simulink model "BEV_Thermal_Management"  (R2025a)
settings: Solver=ode23t  StartTime=0  StopTime=765  MaxStep=5  RelTol=1e-3  AbsTol=1e-3
model workspace: external: MATLAB File BEV_Thermal_Management_param.m (data not in the file)
undefined symbols (not defined in the file): Battery, bulb, cabin_doors_conductivity, cabin_duct_area, cabin_glass_conductivity, cabin_roof_conductivity, cabin_T_init, chiller_area_primary, chiller_N_baffles, chiller_N_tubes, chiller_tube_D, chiller_tube_L, chiller_wall_conductivity, chiller_wall_thickness, compressor_rpm_LUT, condenser_air_area_flow, condenser_air_area_primary, condenser_W, condenser_wall_conductivity, condenser_wall_thickness, coolant_channel_D, coolant_pipe_area, coolant_pipe_D, coolant_T_init, coolant_tank_area, coolant_tank_volume, coolant_valve_D_ratio_max, coolant_valve_D_ratio_min, coolant_valve_displacement, coolant_valve_S_max, cycle, DCDC, Edrive, evaporator_air_area_flow, evaporator_air_area_primary, evaporator_W, evaporator_wall_conductivity, evaporator_wall_thickness, heater_max_power, ModuleType1, outlet, ptc_max_power, pump_speed_max, radiationReflectionShields, radiator_air_area_flow, radiator_air_area_primary, radiator_W, radiator_wall_conductivity, radiator_wall_thickness, refrigerant_alpha_init, refrigerant_pipe_D, transRatio
libraries: fl_lib x264, nesl_utility x91, SimscapeFluids_lib x22, sdl_lib x13, ee_lib x9, nesl_utility_internal x4, slpidlib x3, BatteryProtection x3, batt_lib x2, BatteryCurrentManagement x1, autolibsharedcommon x1, simulink x1
(part 3 of 9)

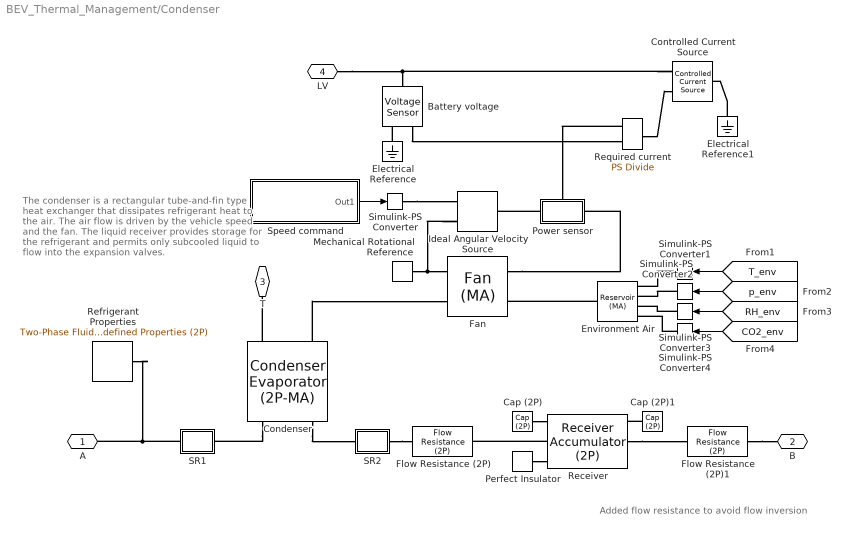
== system BEV_Thermal_Management/Condenser ==
  note: Added flow resistance to avoid flow inversion
  note: The condenser is a rectangular tube-and-fin type heat exchanger that dissipates refrigerant heat to the air. The air flow is driven by the vehicle speed and the fan. The liquid receiver provides storage for the refrigerant and permits only subcooled liquid to flow into the expansion valves.
  Battery voltage : fl_lib/Electrical/Electrical Sensors/Voltage Sensor
  Cap (2P) : fl_lib/Two-Phase Fluid/Elements/Cap (2P)  p_specify=off  p_priority=None  p=0.101325 MPa  p_nominal_specify=off  p_nominal_value=1  p_nominal_unit=MPa  u_specify=off  u_priority=None  u=1.5e+3 kJ/kg  u_nominal_specify=off  u_nominal_value=1  u_nominal_unit=kJ/kg
      settings: InternalSimscapePortConfiguration="{\"Bottom\":[],\"Left\":[{\"id\":\"A\",\"label\":\"\",\"type\":\"foundation.two_phase_fluid.two_phase_fluid\"}],\"Right\":[],\"Top\":[]}"
  Cap (2P)1 : fl_lib/Two-Phase Fluid/Elements/Cap (2P)  p_specify=off  p_priority=None  p=0.101325 MPa  p_nominal_specify=off  p_nominal_value=1  p_nominal_unit=MPa  u_specify=off  u_priority=None  u=1.5e+3 kJ/kg  u_nominal_specify=off  u_nominal_value=1  u_nominal_unit=kJ/kg
      settings: InternalSimscapePortConfiguration="{\"Bottom\":[],\"Left\":[{\"id\":\"A\",\"label\":\"\",\"type\":\"foundation.two_phase_fluid.two_phase_fluid\"}],\"Right\":[],\"Top\":[]}"
  Condenser : SimscapeFluids_lib/Heat Exchangers/Two-Phase Fluid - Moist Air/Condenser Evaporator (2P-MA)  flow_arrangement=fluids.heat_exchangers.enum.FlowArrangement2PMA.Cross  cross_flow_arrangement=fluids.heat_exchangers.enum.CrossFlowArrangement2PMA.UnmixedUnmixed  R_wall=condenser_wall_thickness / condenser_air_area_primary / condenser_wall_conductivity K/W  wall_thermal_mass=false  mass_wall=1 kg  cp_wall=490 J/(K*kg)  area_A1=pi * refrigerant_pipe_D^2 / 4 m^2  area_B1=pi * refrigerant_pipe_D^2 / 4 m^2  area_A2=cabin_duct_area m^2  area_B2=cabin_duct_area m^2  tube_num_2P=condenser_N_tubes  tube_length_2P=condenser_L m  tube_cross_section_2P=fluids.heat_exchangers.enum.TubeCrossSection.Rectangular  tube_diameter_2P=0.1 m  tube_width_2P=condenser_W m  tube_height_2P=condenser_tube_H m  tube_inner_diameter_2P=0.05 m  tube_outer_diameter_2P=0.1 m  tube_flow_area_2P=0.01 m^2  tube_wetted_perimeter_2P=0.4 m  tube_heat_perimeter_2P=0.4 m  tube_pressure_loss_spec_2P=fluids.heat_exchangers.enum.TubePressureLossSpec2P.Haaland  tube_loss_coeff_2P=10  tube_local_pressure_loss_spec_2P=fluids.heat_exchangers.enum.LocalLossSpec.AggregateLength  tube_length_add_2P=condenser_tube_Leq m  tube_local_loss_coefficient_2P=0.1  tube_roughness_pressure_2P=15e-6 m  tube_Re_lam_pressure_2P=2000  tube_Re_tur_pressure_2P=4000  tube_shape_factor_generic_2P=64  tube_heat_coeff_spec_2P=fluids.heat_exchangers.enum.TubeHeatCoeffSpec2P.GneilinskiCavalliniZecchin  tube_colburn_coeff_liq_2P=[.023, .8, .33]  tube_colburn_coeff_mix_2P=[.05, .8, .33]  tube_colburn_coeff_vap_2P=[.023, .8, .33]  tube_roughness_heat_2P=15e-6 m  tube_Re_lam_heat_2P=2000  tube_Re_tur_heat_2P=4000  tube_Nu_lam_generic_2P=3.66  fouling_factor_2P=0.1 m^2*K/kW  fin_area_2P=condenser_tube_area_webs m^2  fin_efficiency_2P=0.6  energy_spec_2P=foundation.enum.energy_spec.void_fraction  p_init_2P=refrigerant_p_init MPa  T_init_2P=293.15 K  x_init_2P=0.5  alpha_init_2P=refrigerant_alpha_init  h_init_2P=1500 kJ/kg  u_init_2P=1500 kJ/kg  flow_geometry_MA=fluids.heat_exchangers.enum.FlowGeometryMA.Generic  tube_num_MA=1  tube_length_MA=5 m  tube_cross_section_MA=fluids.heat_exchangers.enum.TubeCrossSection.Circular  tube_diameter_MA=0.1 m  tube_width_MA=0.1 m  tube_height_MA=0.1 m  tube_inner_diameter_MA=0.05 m  tube_outer_diameter_MA=0.1 m  tube_flow_area_MA=0.01 m^2  tube_wetted_perimeter_MA=0.4 m  tube_heat_perimeter_MA=0.4 m  tube_pressure_loss_spec_MA=fluids.heat_exchangers.enum.TubePressureLossSpec.Haaland  tube_loss_coeff_MA=10  tube_local_pressure_loss_spec_MA=fluids.heat_exchangers.enum.LocalLossSpec.AggregateLength  tube_length_add_MA=0.1 m  tube_local_loss_coefficient_MA=0.1  tube_roughness_pressure_MA=15e-6 m  tube_Re_lam_pressure_MA=2000  tube_Re_tur_pressure_MA=4000  tube_shape_factor_generic_MA=64  tube_heat_coeff_spec_MA=fluids.heat_exchangers.enum.TubeHeatCoeffSpec.Gneilinski  tube_colburn_coeff_MA=[.023, .8, .33]  tube_roughness_heat_MA=15e-6 m  tube_Re_lam_heat_MA=2000  tube_Re_tur_heat_MA=4000  tube_Nu_lam_generic_MA=3.66  bank_arrangement_MA=fluids.heat_exchangers.enum.BankArrangement.Inline  bank_num_rows_MA=5  bank_tubes_per_row_MA=5  bank_width_MA=1 m  bank_tube_diameter_MA=0.05 m  bank_longitudinal_pitch_MA=0.15 m  bank_transverse_pitch_MA=0.15 m  bank_pressure_loss_spec_MA=fluids.heat_exchangers.enum.BankPressureLossSpec.Martin  bank_euler_MA=10  bank_heat_coeff_spec_MA=fluids.heat_exchangers.enum.BankHeatCoeffSpec.Martin  bank_colburn_coeff_MA=[.27, .63, .36]  generic_flow_area_MA=condenser_air_area_flow m^2  generic_heat_area_MA=condenser_air_area_primary m^2  generic_volume_MA=condenser_air_area_flow * condenser_W m^3  generic_loss_coeff_MA=10  generic_colburn_coeff_MA=[0.27, 0.63, 0.36]  fouling_factor_MA=0.1 m^2*K/kW  fin_area_MA=condenser_air_area_fins m^2  fin_efficiency_MA=0.7  p_init_MA=cabin_p_init MPa  T_init_MA=cabin_T_init K  humidity_spec_MA=foundation.enum.HumiditySpec.RelativeHumidity  RH_init_MA=cabin_RH_init  x_w_init_MA=0.01  y_w_init_MA=0.01  HR_init_MA=0.01  Tw_init_MA=287 K  trace_gas_spec_MA=foundation.enum.trace_gas_spec.mole_fraction  x_g_init_MA=0.001  y_g_init_MA=cabin_CO2_init  r_d_init_MA=0  RH_ws_MA=1  time_constant_cond_MA=1e-3 s  time_constant_evap_MA=1e-3 s  fraction_entrained_MA=1
      settings: InternalSimscapePortConfiguration="{\"Bottom\":[],\"Left\":[{\"id\":\"A1\",\"label\":\"A1\",\"type\":\"foundation.two_phase_fluid.two_phase_fluid\"},{\"id\":\"Z\",\"label\":\"Z\",\"type\":\"output\"},{\"id\":\"B1\",\"label\":\"B1\",\"type\":\"foundation.two_phase_fluid.two_phase_fluid\"}],\"Right\":[{\"id\":\"A2\",\"label\":\"A2\",\"type\":\"foundation.moist_air.moist_air\"},{\"id\":\"W\",\"label\":\"W\",\"type\":\"output\"},{\"id\":\"B2\",\"label\":\"B2\",\"type\":\"foundation.moist_air.moist_air\"}],\"Top\":[]}"
  Controlled Current Source : fl_lib/Electrical/Electrical Sources/Controlled Current Source
  Electrical Reference : fl_lib/Electrical/Electrical Elements/Electrical Reference
  Electrical Reference1 : fl_lib/Electrical/Electrical Elements/Electrical Reference
  Environment Air : fl_lib/Moist Air/Elements/Reservoir (MA)  pressure_input=true  pressure_spec=foundation.enum.pressure_spec.atmospheric  reservoir_pressure=0.101325 MPa  temperature_input=true  temperature_spec=foundation.enum.temperature_spec.atmospheric  reservoir_temperature=293.15 K  humidity_input=true  humidity_spec=foundation.enum.HumiditySpec.RelativeHumidity  reservoir_RH=0.5  reservoir_x_w=0.01  reservoir_y_w=0.01  reservoir_HR=0.01  reservoir_Tw=287 K  trace_gas_input=true  trace_gas_spec=foundation.enum.trace_gas_spec.mole_fraction  reservoir_x_g=0.001  reservoir_y_g=0.001  water_droplets_input=false  reservoir_r_d=0  RH_ws=1  area_A=cabin_duct_area m^2  input_error_spec=foundation.enum.input_range_error.warn
      settings: InternalSimscapePortConfiguration="{\"Bottom\":[],\"Left\":[{\"id\":\"A\",\"label\":\"A\",\"type\":\"foundation.moist_air.moist_air\"}],\"Right\":[{\"id\":\"T\",\"label\":\"T\",\"type\":\"input\"},{\"id\":\"P\",\"label\":\"P\",\"type\":\"input\"},{\"id\":\"W\",\"label\":\"W\",\"type\":\"input\"},{\"id\":\"G\",\"label\":\"G\",\"type\":\"input\"}],\"Top\":[]}"
  Fan : SimscapeFluids_lib/Moist Air/Turbomachinery/Fan (MA)  fan_parameterization=fluids.moist_air.turbomachinery.enum.FanParameterization.Nominal  mechanical_power_spec=fluids.moist_air.turbomachinery.enum.FanMechanicalPowerSpec.Efficiency  flow_rate_nominal=0.8 m^3/s  pressure_nominal=400 Pa  eta_nominal=0.6  power_nominal=1620 W  pressure_max=600 Pa  flow_rate_max=1.5 m^3/s  omega_ref_nominal=1000 rpm  flow_rate_1D_TLU=[.0278, .0556, .0833, .111, .139, .167] m^3/s  pressure_1D_TLU=[6410, 6375, 6018, 5366, 4501, 3609] Pa  eta_1D_TLU=[.257, .394, .453, .47, .459, .415]  power_1D_TLU=[693, 900, 1107, 1267, 1363, 1452] W  omega_ref_1D=3000 rpm  rho_ref_1D=1.2 kg/m^3  omega_threshold_factor=1e-2  omega_dp_TLU=[2400; 3000; 3600] rpm  flow_rate_dp_TLU=[.0278, .0556, .0833, .111, .139, .167] m^3/s  pressure_dp_TLU=[4111, 4010, 3551, 2881, 2167, 1453; 6410, 6375, 6018, 5366, 4501, 3609; 9217, 9285, 9022, 8428, 7552, 6482] Pa  eta_dp_TLU=[.3, .434, .468, .459, .4, .3; .257, .394, .453, .47, .459, .415; .225, .359, .434, .461, .47, .459]  power_dp_TLU=[381, 514, 632, 697, 753, 809; 693, 900, 1107, 1267, 1363, 1452; 1139, 1438, 1732, 2029, 2233, 2358] W  rho_ref_dp=1.2 kg/m^3  omega_q_TLU=[2990; 3450; 3867] rpm  pressure_q_TLU=[31, 62, 93, 124] Pa  flow_rate_q_TLU=[.802, .759, .703, .611; .936, .902, .862, .81; 1.056, 1.027, .994, .956] m^3/s  eta_q_TLU=[.088, .162, .22, .261; .068, .128, .18, .222; .055, .105, .148, .188]  power_q_TLU=[283, 290, 297, 290; 427, 437, 445, 452; 595, 606, 625, 631] W  rho_ref_q=1.2 kg/m^3  diameter_ratio=1  mech_orientation=fluids.moist_air.turbomachinery.enum.FanMechanicalOrientation.Positive  area_A=cabin_duct_area m^2  area_B=cabin_duct_area m^2
      settings: InternalSimscapePortConfiguration="{\"Bottom\":[],\"Left\":[{\"id\":\"A\",\"label\":\"A\",\"type\":\"foundation.moist_air.moist_air\"},{\"id\":\"C\",\"label\":\"C\",\"type\":\"foundation.mechanical.rotational.rotational\"}],\"Right\":[{\"id\":\"B\",\"label\":\"B\",\"type\":\"foundation.moist_air.moist_air\"},{\"id\":\"R\",\"label\":\"R\",\"type\":\"foundation.mechanical.rotational.rotational\"}],\"Top\":[]}"
  Flow Resistance (2P) : fl_lib/Two-Phase Fluid/Elements/Flow Resistance (2P)  delta_p_nominal=1e-2 MPa  mdot_nominal=0.01 kg/s  v_nominal=0 m^3/kg  area=pi * refrigerant_pipe_D^2 / 4 m^2  laminar_fraction=1e-3
      settings: InternalSimscapePortConfiguration="{\"Bottom\":[],\"Left\":[{\"id\":\"A\",\"label\":\"A\",\"type\":\"foundation.two_phase_fluid.two_phase_fluid\"}],\"Right\":[{\"id\":\"B\",\"label\":\"B\",\"type\":\"foundation.two_phase_fluid.two_phase_fluid\"}],\"Top\":[]}"
  Flow Resistance (2P)1 : fl_lib/Two-Phase Fluid/Elements/Flow Resistance (2P)  delta_p_nominal=1e-2 MPa  mdot_nominal=0.01 kg/s  v_nominal=0 m^3/kg  area=pi * refrigerant_pipe_D^2 / 4 m^2  laminar_fraction=1e-3
      settings: InternalSimscapePortConfiguration="{\"Bottom\":[],\"Left\":[{\"id\":\"A\",\"label\":\"A\",\"type\":\"foundation.two_phase_fluid.two_phase_fluid\"}],\"Right\":[{\"id\":\"B\",\"label\":\"B\",\"type\":\"foundation.two_phase_fluid.two_phase_fluid\"}],\"Top\":[]}"
  Ideal Angular Velocity Source : fl_lib/Mechanical/Mechanical Sources/Ideal Angular Velocity Source
  Mechanical Rotational Reference : fl_lib/Mechanical/Rotational Elements/Mechanical Rotational Reference
  Perfect Insulator : fl_lib/Thermal/Thermal Elements/Perfect Insulator  T_specify=off  T_priority=None  T=0 K  T_nominal_specify=off  T_nominal_value=1  T_nominal_unit=K
  Power sensor : Subsystem
      settings: PortSchema="{\"entries\":[{\"content\":{\"sides\":[{\"content\":{\"connectorIds\":[\"LConn1\"]},\"type\":\"ConnectorPlacement.EquallySpacedRectSide\",\"uuid\":\"14aacb84-4d2c-4fe3-9667-966fc9affdc2\"},{\"content\":{\"connectorIds\":[\"RConn1\"],\"side\":\"RIGHT\"},\"type\":\"ConnectorPlacement.EquallySpacedRectSide\",\"uuid\":\"5f04cc75-bf75-44ff-ad13-d2b18990cf19\"},{\"content\":{\"connectorIds\":[\"LConn2\"],\"side\":\"TOP\"},\"type\":\"ConnectorPlacement.EquallySpacedRectSide\",\"uuid\":\"fdf9b4dd-6b03-4f92-a45a-c9cb867bd95a\"}]},\"type\":\"ConnectorPlacement.EquallySpacedConnector\",\"uuid\":\"3effddba-6f65-4497-8868-e18a0983ff0c\"}],\"packageUris\":[\"http://schema.mathworks.com/mf0/Connector/R2020b\"],\"version\":\"1.0\"}"
  Receiver : SimscapeFluids_lib/Two-Phase Fluid/Tanks & Accumulators/Receiver Accumulator (2P)  volume=2 l  tank_area=0.5 m^2  area_AV=0.01 m^2  area_BV=0.01 m^2  area_AL=pi * refrigerant_pipe_D^2 / 4 m^2  area_BL=pi * refrigerant_pipe_D^2 / 4 m^2  V_frac_liq_error=simscape.enum.assert.action.none  V_frac_liq_min=0.05  V_frac_liq_max=0.95  V_frac_smooth=0.05  p_crit_error=simscape.enum.assert.action.error  hc_vap=20 W/(m^2*K)  hc_liq=100 W/(m^2*K)  p_init=refrigerant_p_init MPa  fraction_spec=fluids.two_phase_fluid.tanks_accumulators.enum.LiquidFractionSpec.Volume  M_frac_liq_init=0.5  V_frac_liq_init=1 - refrigerant_alpha_init  saturated_init=true  energy_spec=fluids.two_phase_fluid.tanks_accumulators.enum.EnergySpec.SubcoolingSuperheating  delta_T_sub_init=5 deltaK  delta_T_sup_init=5 deltaK  T_liq_init=368.15 K  T_vap_init=378.15 K  h_liq_init=400 kJ/kg  h_vap_init=2700 kJ/kg  u_liq_init=400 kJ/kg  u_vap_init=2700 kJ/kg  tau_vap_cond=1 s
      settings: InternalSimscapePortConfiguration="{\"Bottom\":[],\"Left\":[{\"id\":\"AV\",\"label\":\"AV\",\"type\":\"foundation.two_phase_fluid.two_phase_fluid\"},{\"id\":\"AL\",\"label\":\"AL\",\"type\":\"foundation.two_phase_fluid.two_phase_fluid\"},{\"id\":\"H\",\"label\":\"H\",\"type\":\"foundation.thermal.thermal\"}],\"Right\":[{\"id\":\"BV\",\"label\":\"BV\",\"type\":\"foundation.two_phase_fluid.two_phase_fluid\"},{\"id\":\"BL\",\"label\":\"BL\",\"type\":\"foundation.two_phase_fluid.two_phase_fluid\"},{\"id\":\"L\",\"label\":\"L\",\"type\":\"output\"}],\"Top\":[]}"
  Refrigerant Properties : SimscapeFluids_lib/Two-Phase Fluid/Utilities/Two-Phase Fluid Predefined Properties (2P)  fluid=fluids.two_phase_fluid.utilities.enum.Fluid.R134a  p_atm=0.101325 MPa  properties_range_check=simscape.enum.assert.action.error  q_rev=0.01 Pa
  Required current : fl_lib/Physical Signals/Functions/PS Divide
  SR1 : Subsystem
      mask Display: disp(get_param(gcb, 'Name'))
  SR2 : Subsystem
      mask Display: disp(get_param(gcb, 'Name'))
  Simulink-PS Converter : nesl_utility/Simulink-PS Converter  PhysicalDomain=network_engine_domain  SubClassName=ps_input  LeftPortType=input  RightPortType=output  PseudoPeriodic=off  Frequencies=[]  NoiseDistribution=none  NoiseParameters=[]  Unit=rpm  AffineConversion=off  FilteringAndDerivatives=provide  SimscapeFilterOrder=1  InputFilterTimeConstant=0.001  UdotUserProvided=0
  Simulink-PS Converter1 : nesl_utility/Simulink-PS Converter  PhysicalDomain=network_engine_domain  SubClassName=ps_input  LeftPortType=input  RightPortType=output  PseudoPeriodic=off  Frequencies=[]  NoiseDistribution=none  NoiseParameters=[]  Unit=degC  AffineConversion=on  FilteringAndDerivatives=provide  SimscapeFilterOrder=1  InputFilterTimeConstant=0.001  UdotUserProvided=0
  Simulink-PS Converter2 : nesl_utility/Simulink-PS Converter  PhysicalDomain=network_engine_domain  SubClassName=ps_input  LeftPortType=input  RightPortType=output  PseudoPeriodic=off  Frequencies=[]  NoiseDistribution=none  NoiseParameters=[]  Unit=MPa  AffineConversion=off  FilteringAndDerivatives=provide  SimscapeFilterOrder=1  InputFilterTimeConstant=0.001  UdotUserProvided=0
  Simulink-PS Converter3 : nesl_utility/Simulink-PS Converter  PhysicalDomain=network_engine_domain  SubClassName=ps_input  LeftPortType=input  RightPortType=output  PseudoPeriodic=off  Frequencies=[]  NoiseDistribution=none  NoiseParameters=[]  Unit=1  AffineConversion=off  FilteringAndDerivatives=provide  SimscapeFilterOrder=1  InputFilterTimeConstant=0.001  UdotUserProvided=0
  Simulink-PS Converter4 : nesl_utility/Simulink-PS Converter  PhysicalDomain=network_engine_domain  SubClassName=ps_input  LeftPortType=input  RightPortType=output  PseudoPeriodic=off  Frequencies=[]  NoiseDistribution=none  NoiseParameters=[]  Unit=1  AffineConversion=off  FilteringAndDerivatives=provide  SimscapeFilterOrder=1  InputFilterTimeConstant=0.001  UdotUserProvided=0
  Speed command : Subsystem
      mask Display: disp('Speed command')
  A : PMIOPort  Side=Left
  B : PMIOPort  Port=2  Side=Left
  T : PMIOPort  Port=3  Side=Left
  LV : PMIOPort  Port=4  Side=Right
  wires:
  [T_env] -> Simulink-PS Converter1/1
  [p_env] -> Simulink-PS Converter2/1
  [RH_env] -> Simulink-PS Converter3/1
  [CO2_env] -> Simulink-PS Converter4/1
  Speed command/1(Out1) -> Simulink-PS Converter/1
  connections:
  Condenser/LConn1 -- SR1/RConn1
  Condenser/LConn3 -- SR2/LConn1
  Receiver/LConn2 -- Flow Resistance (2P)/RConn1
  Cap (2P)/LConn1 -- Receiver/LConn1
  Cap (2P)1/LConn1 -- Receiver/RConn1
  Condenser/RConn1 -- T/RConn1
  Simulink-PS Converter2/RConn1 -- Environment Air/RConn2
  Simulink-PS Converter4/RConn1 -- Environment Air/RConn4
  Simulink-PS Converter3/RConn1 -- Environment Air/RConn3
  Simulink-PS Converter1/RConn1 -- Environment Air/RConn1
  Environment Air/LConn1 -- Fan/RConn1
  Condenser/RConn3 -- Fan/LConn1
  Perfect Insulator/LConn1 -- Receiver/LConn3
  SR1/LConn1 -- Refrigerant Properties/RConn1 -- A/RConn1
  SR2/RConn1 -- Flow Resistance (2P)/LConn1
  Receiver/RConn2 -- Flow Resistance (2P)1/LConn1
  Ideal Angular Velocity Source/RConn2 -- Mechanical Rotational Reference/LConn1 -- Fan/LConn2
  Simulink-PS Converter/RConn1 -- Ideal Angular Velocity Source/RConn1
  Power sensor/LConn1 -- Ideal Angular Velocity Source/LConn1
  Fan/RConn2 -- Power sensor/RConn1
  LV/RConn1 -- Battery voltage/LConn1 -- Controlled Current Source/RConn2
  Required current/LConn1 -- Power sensor/LConn2
  Required current/RConn1 -- Controlled Current Source/RConn1
  Battery voltage/RConn1 -- Required current/LConn2
  Electrical Reference/LConn1 -- Battery voltage/RConn2
  Electrical Reference1/LConn1 -- Controlled Current Source/LConn1
  Flow Resistance (2P)1/RConn1 -- B/RConn1

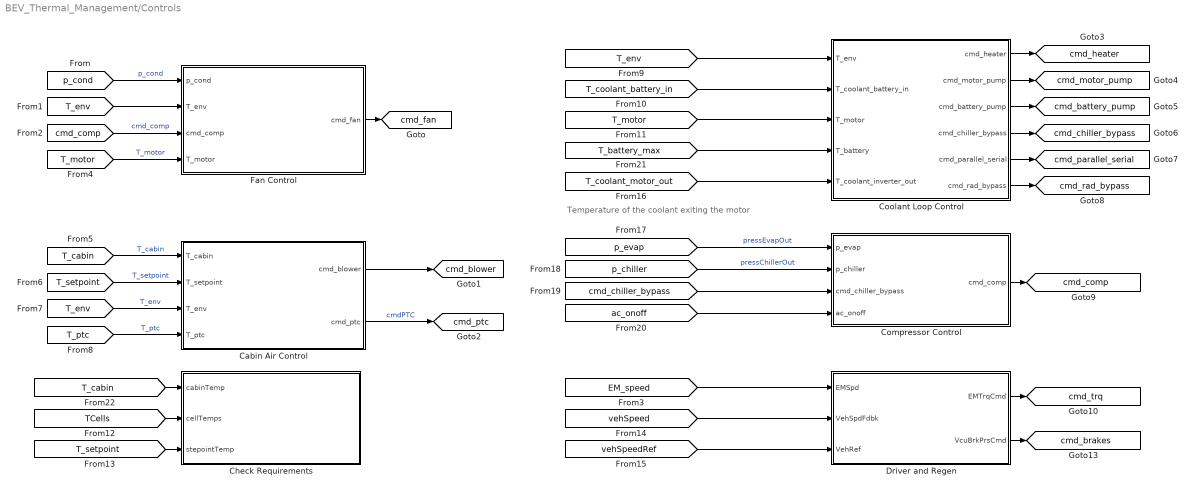
== system BEV_Thermal_Management/Controls ==
  note: Temperature of the coolant exiting the motor
  Cabin Air Control : Subsystem
      mask Display: disp('Cabin\nAir\nControl')
  Check Requirements : Subsystem
  Compressor Control : Subsystem
  Coolant Loop Control : Subsystem
  Driver and Regen : Subsystem
      mask Display: disp('Driver and Regen')
  Fan Control : Subsystem
      mask Display: disp('Fan\nControl')
  tag scope: cmd_battery_pump=global, cmd_blower=global, cmd_brakes=global, cmd_chiller_bypass=global, cmd_comp=global, cmd_fan=global, cmd_heater=global, cmd_motor_pump=global, cmd_parallel_serial=global, cmd_ptc=global, cmd_rad_bypass=global, cmd_trq=global
  wires:
  [p_cond] -> Fan Control/1(p_cond)  "p_cond"
  [T_env] -> Fan Control/2(T_env)
  [T_motor] -> Fan Control/4(T_motor)  "T_motor"
  [T_env] -> Coolant Loop Control/1(T_env)
  [T_coolant_battery_in] -> Coolant Loop Control/2(T_coolant_battery_in)
  Fan Control/1(cmd_fan) -> [cmd_fan]
  Coolant Loop Control/1(cmd_heater) -> [cmd_heater]
  Coolant Loop Control/2(cmd_motor_pump) -> [cmd_motor_pump]
  Coolant Loop Control/3(cmd_battery_pump) -> [cmd_battery_pump]
  [p_evap] -> Compressor Control/1(p_evap)  "pressEvapOut"
  [p_chiller] -> Compressor Control/2(p_chiller)  "pressChillerOut"
  [cmd_chiller_bypass] -> Compressor Control/3(cmd_chiller_bypass)
  [ac_onoff] -> Compressor Control/4(ac_onoff)
  Compressor Control/1(cmd_comp) -> [cmd_comp]
  Cabin Air Control/1(cmd_blower) -> [cmd_blower]
  Cabin Air Control/2(cmd_ptc) -> [cmd_ptc]  "cmdPTC"
  Coolant Loop Control/4(cmd_chiller_bypass) -> [cmd_chiller_bypass]
  Coolant Loop Control/5(cmd_parallel_serial) -> [cmd_parallel_serial]
  Coolant Loop Control/6(cmd_rad_bypass) -> [cmd_rad_bypass]
  [T_motor] -> Coolant Loop Control/3(T_motor)
  [T_coolant_motor_out] -> Coolant Loop Control/5(T_coolant_inverter_out)
  [cmd_comp] -> Fan Control/3(cmd_comp)  "cmd_comp"
  [T_cabin] -> Cabin Air Control/1(T_cabin)  "T_cabin"
  [T_setpoint] -> Cabin Air Control/2(T_setpoint)  "T_setpoint"
  [T_env] -> Cabin Air Control/3(T_env)  "T_env"
  [T_ptc] -> Cabin Air Control/4(T_ptc)  "T_ptc"
  [T_battery_max] -> Coolant Loop Control/4(T_battery)
  [EM_speed] -> Driver and Regen/1(EMSpd)
  Driver and Regen/1(EMTrqCmd) -> [cmd_trq]
  Driver and Regen/2(VcuBrkPrsCmd) -> [cmd_brakes]
  [vehSpeed] -> Driver and Regen/2(VehSpdFdbk)
  [vehSpeedRef] -> Driver and Regen/3(VehRef)
  [T_cabin] -> Check Requirements/1(cabinTemp)
  [TCells] -> Check Requirements/2(cellTemps)
  [T_setpoint] -> Check Requirements/3(stepointTemp)

== system BEV_Thermal_Management/DCDC ==
  note: Electrical Model
  note: Thermal Model
  note: This subsystem models a coolant jacket around the DC-DC converter, which is represented by a heat flow rate source and a thermal mass.
      | The DCDC system connects the HV side of the battery to the LV side of the pumps
  Convective Heat Transfer : fl_lib/Thermal/Thermal Elements/Convective Heat Transfer  thermal_type=foundation.enum.constant_variable.constant  area=3e-5 m^2  heat_tr_coeff=5 W/(K*m^2)  min_heat_tr_coeff=1e-3 W/(K*m^2)  T_specify=off  T_priority=None  T=0 K  T_nominal_specify=off  T_nominal_value=1  T_nominal_unit=K  Q_specify=off  Q_priority=None  Q=0 W  Q_nominal_specify=off  Q_nominal_value=1  Q_nominal_unit=W
  Coolant Jacket : SimscapeFluids_lib/Thermal Liquid/Pipes & Fittings/Pipe (TL)  dynamic_compressibility=simscape.enum.onoff.on  inertia=simscape.enum.onoff.off  num_segments=1  pipe_length=0.2 m  cross_section_geometry=fluids.thermal_liquid.pipes_fittings.enum.CrossSectionGeometry.Custom  pipe_diameter=0.1 m  pipe_inner_diameter=0.05 m  pipe_outer_diameter=0.1 m  pipe_width=0.1 m  pipe_height=0.1 m  pipe_major_axis=0.1 m  pipe_minor_axis=0.05 m  pipe_side=0.1 m  pipe_angle=30 deg  area=pi * coolant_channel_D^2 / 4 m^2  Dh=coolant_channel_D m  elevation_spec=foundation.enum.constant_variable.constant  elevation_gain=0 m  gravity_spec=foundation.enum.constant_variable.constant  g=9.81 m/s^2  pressure_loss_spec=fluids.thermal_liquid.pipes_fittings.enum.PressureLossSpec.Haaland  local_pressure_loss_spec=fluids.thermal_liquid.pipes_fittings.enum.LocalLossSpec.AggregateLength  length_add=0 m  loss_coefficient=0.1  roughness_spec=fluids.thermal_liquid.pipes_fittings.enum.RoughnessSpec.Custom  roughness=1.5e-5 m  Re_friction_TLU=[ 400 1000 1.5e+3 3e+3 4e+3 6e+3 1e+4 2e+4 4e+4 6e+4 1e+5 1e+8 ]  friction_factor_TLU=[ 0.264 0.112 0.07099999999999999 0.0417 0.0387 0.0268 0.025 0.0232 0.0226 0.022 0.0214 0.0214 ]  Re_lam=100  Re_tur=500  shape_factor=64  mdot_nominal=[ 0.1 1 ] kg/s  p_diff_nominal=[ 0.001 0.01 ] MPa  mdot_threshold=1e-6 kg/s  wall_spec=fluids.thermal_liquid.pipes_fittings.enum.wall_spec.rigid  vol_expansion_spec=fluids.thermal_liquid.pipes_fittings.enum.VolumeExpansionSpec.Diameter  area_pressure_gain=1e-6 m^2/MPa  static_pressure_TLU=[.1, 1] MPa  area_pressure_gain_TLU=[1e-05, 1.1e-05] m^2  material_behavior_spec=fluids.thermal_liquid.pipes_fittings.enum.PipeMaterialBehavior.Linear  diameter_pressure_gain=1.2e-6 m/MPa  wall_thickness=0.05 m  elastic_modulus=69 GPa  stress_TLU=[276, 310] MPa  strain_TLU=[.004, .02]  stress_assert_action=simscape.enum.assert.action.none  stress_max=400 MPa  poisson_ratio=0.33  wall_time_constant=0.01 s  thermal_expansion=false  alpha_L_wall=24 um/(deltaK*m)  thermal_expansion_Tref=293.15 K  heat_transfer_spec=fluids.thermal_liquid.pipes_fittings.enum.HeatTransferSpec.DittusBoelter  mdot_nominal_heat=[ 0.1 1 ] kg/s  T_in_nominal=[ 293.15 293.15 ] K  T_out_nominal=[ 300 300 ] K  p_in_nominal_heat=[ 0.101325 0.101325 ] MPa  T_wall_nominal=[ 303.15 303.15 ] K  a_coeff=0.3  b_Re_power=0.8  c_Pr_power=0.33  Nu_lam=3.66  Re_Colburn_TLU=[ 100 150 1000 ]  Colburn_factor_TLU=[ 0.019 0.013 0.002 ]  Re_Nu_TLU=[ 100 150 1000 ]  Pr_Nu_TLU=[ 1 10 ]  Nu_TLU=[ 3.72 4.21; 3.75 4.44; 4.21 7.15 ]  p0_vec=coolant_p_init MPa  T0_vec=coolant_T_init K  mdot0=0.1 kg/s  p_nominal=0.101325 MPa  T_nominal=293.15 K
  "DCDC " : ee_lib/Semiconductors & Converters/Converters/DC-DC Converter  Vref_option=ee.enum.converters.voltageref.internal  v_ref="DCDC.DCDCOutputVltg  V"  P_rated=DCDC.DCRatedPwr W  droop_enabled=false  droop_param=ee.enum.converters.droop.value  droop=0.1 V/A  droop_percent=2  Vref_droop=10 V  reversible=ee.enum.converters.directionality.unidirectional  G_diode=1e-8 1/Ohm  P_fixed=100 W  losses_option=ee.enum.converters.lossesOption.proportionalToSquaredCurrent  eff_rated=DCDC.DCDCEff*100  tableOption=ee.enum.converters.lossTableOptionThermal.currentTemp  i_eff_vec=[-2, -1, 1, 2] A  v_eff_vec=[15, 30, 45] V  eff_vec=[66, 76, 80, 74]  eff_2D_table=[66, 66, 66; 76, 76, 76; 80, 80, 80; 74, 74, 74]  model_dynamics=ee.enum.converters.dynamics.yes  tau=0.02 s  v_ini=12 V  v1_min=1 V  R1=1000 Ohm  R2=1000 Ohm  fault_condition=ee.enum.faults.faultInputCondition.greaterThan  fault_threshold=0.5  T_eff_vec=[280, 300, 320] K  eff_3D_table=repmat([66; 76; 80; 74], 1, 3, 3)  thermal_mass=4000 J/K  initial_temperature=coolant_T_init K
      settings: InternalSimscapePortConfiguration="{\"Bottom\":[],\"Left\":[{\"id\":\"p1\",\"label\":\"1+\",\"type\":\"foundation.electrical.electrical\"},{\"id\":\"n1\",\"label\":\"1-\",\"type\":\"foundation.electrical.electrical\"}],\"Right\":[{\"id\":\"p2\",\"label\":\"2+\",\"type\":\"foundation.electrical.electrical\"},{\"id\":\"n2\",\"label\":\"2-\",\"type\":\"foundation.electrical.electrical\"},{\"id\":\"H\",\"label\":\"H\",\"type\":\"foundation.thermal.thermal\"}],\"Top\":[]}"
  Electrical Reference : fl_lib/Electrical/Electrical Elements/Electrical Reference
  Electrical Reference1 : fl_lib/Electrical/Electrical Elements/Electrical Reference
  Environment Temperature : fl_lib/Thermal/Thermal Sources/Controlled Temperature Source
  Flow Resistance (TL) : fl_lib/Thermal Liquid/Elements/Flow Resistance (TL)  delta_p_nominal=2e-3 MPa  mdot_nominal=0.02 kg/s  area=coolant_pipe_area m^2  laminar_fraction=1e-3
  Flow Resistance (TL)1 : fl_lib/Thermal Liquid/Elements/Flow Resistance (TL)  delta_p_nominal=1e-5 MPa  mdot_nominal=0.02 kg/s  area=coolant_pipe_area m^2  laminar_fraction=1e-3
  Heat Conduction Housing In : fl_lib/Thermal/Thermal Elements/Conductive Heat Transfer  thermal_type=foundation.enum.ConstantVariableTabulated.Constant  wall_geometry=foundation.enum.ConductionWallGeometry.Planar  area=3e-5 m^2  thickness=0.005 m  d_in=Edrive.diameter-0.005 m  d_out=Edrive.diameter m  L=Edrive.length m  th_cond_min=10 W/(K*m)  th_cond=230 W/(K*m)  th_cond_TLU=[413, 401, 392, 383, 371, 357, 342] W/(K*m)  temp_TLU=[200, 273, 400, 600, 800, 1000, 1200] K  T_specify=off  T_priority=None  T=0 K  T_nominal_specify=off  T_nominal_value=1  T_nominal_unit=K  Q_specify=off  Q_priority=None  Q=0 W  Q_nominal_specify=off  Q_nominal_value=1  Q_nominal_unit=W
  Heat Conduction Housing Out : fl_lib/Thermal/Thermal Elements/Conductive Heat Transfer  thermal_type=foundation.enum.ConstantVariableTabulated.Constant  wall_geometry=foundation.enum.ConductionWallGeometry.Planar  area=3e-5 m^2  thickness=0.005 m  d_in=Edrive.diameter-0.005 m  d_out=Edrive.diameter m  L=Edrive.length m  th_cond_min=10 W/(K*m)  th_cond=230 W/(K*m)  th_cond_TLU=[413, 401, 392, 383, 371, 357, 342] W/(K*m)  temp_TLU=[200, 273, 400, 600, 800, 1000, 1200] K  T_specify=off  T_priority=None  T=0 K  T_nominal_specify=off  T_nominal_value=1  T_nominal_unit=K  Q_specify=off  Q_priority=None  Q=0 W  Q_nominal_specify=off  Q_nominal_value=1  Q_nominal_unit=W
  Housing : fl_lib/Thermal/Thermal Elements/Thermal Mass  mass_type=foundation.enum.constant_variable.constant  mass=2 kg  sp_heat=900 J/(K*kg)  mass_min=1e-6 kg  num_ports=foundation.enum.numPorts2.one  m_specify=off  m_priority=High  m=1 kg  m_nominal_specify=off  m_nominal_value=1  m_nominal_unit=kg  T_specify=on  T_priority=High  T=coolant_T_init K  T_nominal_specify=off  T_nominal_value=1  T_nominal_unit=K  Q_specify=off  Q_priority=None  Q=0 W  Q_nominal_specify=off  Q_nominal_value=1  Q_nominal_unit=W
  PS-Simulink Converter : nesl_utility/PS-Simulink Converter  PhysicalDomain=network_engine_domain  SubClassName=ps_output  LeftPortType=input  RightPortType=output  PseudoPeriodic=off  Frequencies=[]  VectorFormat=1-D array  Unit=degC  AffineConversion=on
  PWRS7 : Subsystem
      mask Display: disp(get_param(gcb,'Name'))
  PWRS8 : Subsystem
      mask Display: disp(get_param(gcb,'Name'))
  Resistor : fl_lib/Electrical/Electrical Elements/Resistor  R=1e-6 Ohm  i_specify=on  i_priority=Low  i=0 A  i_nominal_specify=off  i_nominal_value=1  i_nominal_unit=A  v_specify=off  v_priority=None  v=0 V  v_nominal_specify=off  v_nominal_value=1  v_nominal_unit=V
  SC8 : Subsystem
      mask Display: disp(get_param(gcb, 'Name'))
  SC9 : Subsystem
      mask Display: disp(get_param(gcb, 'Name'))
  Simulink-PS Converter2 : nesl_utility/Simulink-PS Converter  PhysicalDomain=network_engine_domain  SubClassName=ps_input  LeftPortType=input  RightPortType=output  PseudoPeriodic=off  Frequencies=[]  NoiseDistribution=none  NoiseParameters=[]  Unit=degC  AffineConversion=on  FilteringAndDerivatives=provide  SimscapeFilterOrder=1  InputFilterTimeConstant=0.001  UdotUserProvided=0
  Temperature Sensor : fl_lib/Thermal/Thermal Sensors/Temperature Sensor  temperature_measure=foundation.enum.MeasurementReference.difference
  Thermal Reference : fl_lib/Thermal/Thermal Elements/Thermal Reference
  Thermal Reference1 : fl_lib/Thermal/Thermal Elements/Thermal Reference
  B : PMIOPort  Side=Left
  LV : PMIOPort  Port=2  Side=Left
  A : PMIOPort  Port=3  Side=Right
  HV : PMIOPort  Port=4  Side=Right
  tag scope: T_dcdc=global
  wires:
  PS-Simulink Converter/1 -> [T_dcdc]
  [T_env] -> Simulink-PS Converter2/1
  connections:
  "DCDC "/LConn2 -- Electrical Reference/LConn1
  PWRS7/RConn1 -- "DCDC "/LConn1
  LV/RConn1 -- PWRS8/RConn1
  Electrical Reference1/LConn1 -- "DCDC "/RConn2
  "DCDC "/RConn3 -- Heat Conduction Housing In/LConn1 -- Temperature Sensor/LConn1
  Flow Resistance (TL)1/RConn1 -- SC8/LConn1
  Thermal Reference1/LConn1 -- Temperature Sensor/RConn1
  Coolant Jacket/LConn1 -- Flow Resistance (TL)/RConn1
  Temperature Sensor/RConn2 -- PS-Simulink Converter/LConn1
  A/RConn1 -- SC9/LConn1
  Coolant Jacket/RConn1 -- Flow Resistance (TL)1/LConn1
  HV/RConn1 -- PWRS7/LConn1
  PWRS8/LConn1 -- Resistor/RConn1
  Heat Conduction Housing In/RConn1 -- Heat Conduction Housing Out/LConn1 -- Housing/LConn1
  Simulink-PS Converter2/RConn1 -- Environment Temperature/RConn1
  Coolant Jacket/LConn2 -- Convective Heat Transfer/LConn1 -- Heat Conduction Housing Out/RConn1
  Convective Heat Transfer/RConn1 -- Environment Temperature/LConn1
  Thermal Reference/LConn1 -- Environment Temperature/RConn2
  Resistor/LConn1 -- "DCDC "/RConn1
  SC9/RConn1 -- Flow Resistance (TL)/LConn1
  SC8/RConn1 -- B/RConn1

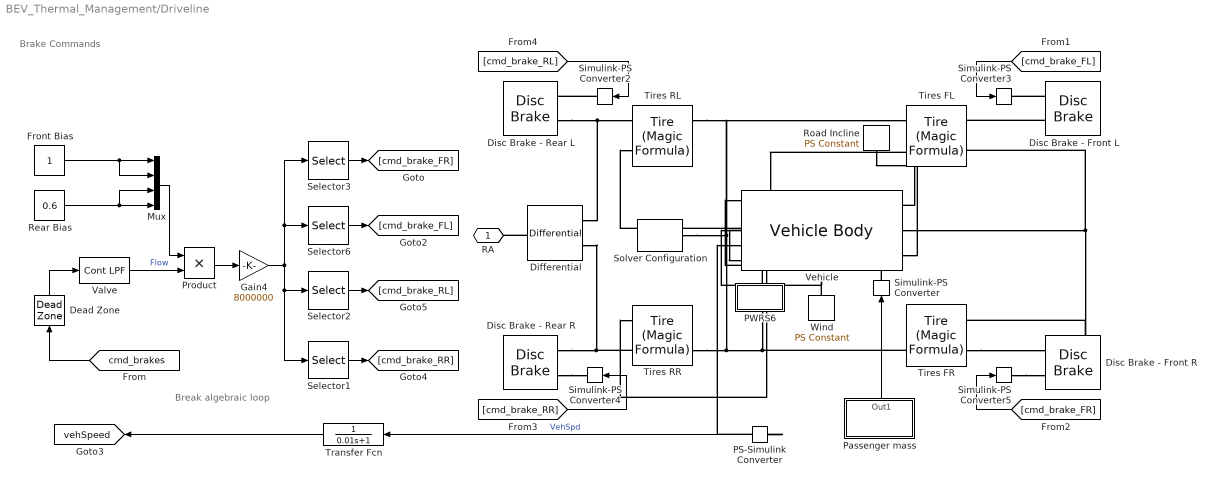
== system BEV_Thermal_Management/Driveline ==
  note: Brake Commands
  note: Break algebraic loop
  Dead Zone : DeadZone  LowerValue=-inf  UpperValue=1e-3  ZeroCross=off
  Differential : sdl_lib/Gears/Differential  driveshaft_location=sdl.enum.differential_orientation.right  cd_ratio=1  friction_model=sdl.enum.gear_friction.none  efficiency=[.85, .92]  temperature_TLU=[280, 300, 320] K  efficiency_ss_TLU=[.95, .9, .85]  efficiency_cd_TLU=[.95, .9, .85]  pwr_thr=[.001, .001] W  mu_visc=[0, 0] N*m*s/rad  model_inertia=simscape.enum.onoff.off  sun_inertia=1e-10 kg*m^2  sun_radius=0.01 m  carrier_inertia=0.001 kg*m^2  planet_inertia=0.001 kg*m^2  planet_mass=1e-10 kg  thermal_mass=50 J/K  T_init=300 K
  Disc Brake - Front L : sdl_lib/Brakes & Detents/Rotational/Disc Brake  r_mean=0.15 m  bore=0.05 m  n_pads=2  thermal_port=simscape.enum.thermaleffects.omit  mu_static=0.45  mu_coulomb=0.35  temperature_TLU=[280, 300, 320] K  mu_static_TLU=[.9, .8, .7]  mu_coulomb_TLU=[.8, .7, .6]  brkwy_vel=0.1 rad/s  visc_coef=0 N*m*s/rad  thermal_mass=50 kJ/K  temperature_specify=off  temperature_priority=High  temperature=300 K  temperature_nominal_specify=off  temperature_nominal_value=1  temperature_nominal_unit=K
  Disc Brake - Front R : sdl_lib/Brakes & Detents/Rotational/Disc Brake  r_mean=0.15 m  bore=0.05 m  n_pads=2  thermal_port=simscape.enum.thermaleffects.omit  mu_static=0.45  mu_coulomb=0.35  temperature_TLU=[280, 300, 320] K  mu_static_TLU=[.9, .8, .7]  mu_coulomb_TLU=[.8, .7, .6]  brkwy_vel=0.1 rad/s  visc_coef=0 N*m*s/rad  thermal_mass=50 kJ/K  temperature_specify=off  temperature_priority=High  temperature=300 K  temperature_nominal_specify=off  temperature_nominal_value=1  temperature_nominal_unit=K
  Disc Brake - Rear L : sdl_lib/Brakes & Detents/Rotational/Disc Brake  r_mean=0.15 m  bore=0.05 m  n_pads=2  thermal_port=simscape.enum.thermaleffects.omit  mu_static=0.45  mu_coulomb=0.35  temperature_TLU=[280, 300, 320] K  mu_static_TLU=[.9, .8, .7]  mu_coulomb_TLU=[.8, .7, .6]  brkwy_vel=0.1 rad/s  visc_coef=0 N*m*s/rad  thermal_mass=50 kJ/K  temperature_specify=off  temperature_priority=High  temperature=300 K  temperature_nominal_specify=off  temperature_nominal_value=1  temperature_nominal_unit=K
  Disc Brake - Rear R : sdl_lib/Brakes & Detents/Rotational/Disc Brake  r_mean=0.15 m  bore=0.05 m  n_pads=2  thermal_port=simscape.enum.thermaleffects.omit  mu_static=0.45  mu_coulomb=0.35  temperature_TLU=[280, 300, 320] K  mu_static_TLU=[.9, .8, .7]  mu_coulomb_TLU=[.8, .7, .6]  brkwy_vel=0.1 rad/s  visc_coef=0 N*m*s/rad  thermal_mass=50 kJ/K  temperature_specify=off  temperature_priority=High  temperature=300 K  temperature_nominal_specify=off  temperature_nominal_value=1  temperature_nominal_unit=K
  Front Bias : Constant  SampleTime=-1
  Gain4 : Gain  Gain=8000000
  Mux : Mux
  PS-Simulink Converter : nesl_utility/PS-Simulink Converter  PhysicalDomain=network_engine_domain  SubClassName=ps_output  LeftPortType=input  RightPortType=output  PseudoPeriodic=off  Frequencies=[]  VectorFormat=inherit  Unit=km/hr  AffineConversion=off
  PWRS6 : Subsystem
      settings: PortSchema="{\"entries\":[{\"content\":{\"sides\":[{\"content\":{},\"type\":\"ConnectorPlacement.EquallySpacedRectSide\",\"uuid\":\"fcd324e3-e0dc-4621-a170-27ec71c6ea26\"},{\"content\":{\"side\":\"RIGHT\"},\"type\":\"ConnectorPlacement.EquallySpacedRectSide\",\"uuid\":\"5064daf2-a26e-4e75-b2a2-eb5e9c9164b2\"},{\"content\":{\"connectorIds\":[\"LConn1\"],\"side\":\"TOP\"},\"type\":\"ConnectorPlacement.EquallySpacedRectSide\",\"uuid\":\"a278b99a-a5a6-4103-93f8-5a35ed8d5e9c\"},{\"content\":{\"connectorIds\":[\"RConn1\"],\"side\":\"BOTTOM\"},\"type\":\"ConnectorPlacement.EquallySpacedRectSide\",\"uuid\":\"392744ff-7f36-4ddc-9af8-a9b1b363187c\"}]},\"type\":\"ConnectorPlacement.EquallySpacedConnector\",\"uuid\":\"5c1b708f-9083-48c2-9497-eb967c2df4ff\"}],\"packageUris\":[\"http://schema.mathworks.com/mf0/Connector/R2020b\"],\"version\":\"1.0\"}"
      mask Display: disp(get_param(gcb,'Name'));
  Passenger mass : Subsystem
      settings: PortSchema="{\"entries\":[{\"content\":{\"sides\":[{\"content\":{},\"type\":\"ConnectorPlacement.EquallySpacedRectSide\",\"uuid\":\"5a596c41-77e2-4acf-9482-89fe05f9a774\"},{\"content\":{\"side\":\"RIGHT\"},\"type\":\"ConnectorPlacement.EquallySpacedRectSide\",\"uuid\":\"d52f72ae-d2bf-411c-988f-deade7e80142\"},{\"content\":{\"connectorIds\":[\"Out1\"],\"side\":\"TOP\"},\"type\":\"ConnectorPlacement.EquallySpacedRectSide\",\"uuid\":\"9f72a4ad-40b2-460c-94c1-3ba2851858c5\"}]},\"type\":\"ConnectorPlacement.EquallySpacedConnector\",\"uuid\":\"83f953f8-a501-422f-8169-4e865cfd3487\"}],\"packageUris\":[\"http://schema.mathworks.com/mf0/Connector/R2020b\"],\"version\":\"1.0\"}"
      mask Display: disp('Passenger\nmass')
  Product : Product
  Rear Bias : Constant  Value=0.6  SampleTime=-1
  Road Incline : fl_lib/Physical Signals/Sources/PS Constant  constant=0
  Selector1 : Selector  InputPortWidth=4  IndexOptions=Index vector (dialog)  Indices=[4]  OutputSizes=1
  Selector2 : Selector  InputPortWidth=4  IndexOptions=Index vector (dialog)  Indices=[3]  OutputSizes=1
  Selector3 : Selector  InputPortWidth=4  IndexOptions=Index vector (dialog)  Indices=[2]  OutputSizes=1
  Selector6 : Selector  InputPortWidth=4  IndexOptions=Index vector (dialog)  Indices=[1]  OutputSizes=1
  Simulink-PS Converter : nesl_utility/Simulink-PS Converter  PhysicalDomain=network_engine_domain  SubClassName=ps_input  LeftPortType=input  RightPortType=output  PseudoPeriodic=off  Frequencies=[]  NoiseDistribution=none  NoiseParameters=[]  Unit=kg  AffineConversion=off  FilteringAndDerivatives=provide  SimscapeFilterOrder=1  InputFilterTimeConstant=0.001  UdotUserProvided=0
  Simulink-PS Converter{2..5} (4 alike) : nesl_utility_internal/Simulink-PS Converter  PhysicalDomain=network_engine_domain  SubClassName=ps_input  LeftPortType=input  RightPortType=output  PseudoPeriodic=off  Frequencies=[]  NoiseDistribution=none  NoiseParameters=[]  Unit=Pa  AffineConversion=off  FilteringAndDerivatives=provide  SimscapeFilterOrder=1  InputFilterTimeConstant=0.001  UdotUserProvided=0
  Solver Configuration : nesl_utility/Solver Configuration  PhysicalDomain=network_engine_domain  SubClassName=solver  LeftPortType=input  RightPortType=generic  Tones=[]  Harmonics=[]  SimulateNoise=off  Profile=off  UseLocalSampling=off  EnableSwitchedLinearOptims=on  FrequencyDomain=off  UseCCode=off  RelTol=0.001  AbsTol=1e-06  MinStep=1e-09  ToWorkspace=off  RevertToSquareIcSolve=off  NumHomotopyIterations=100  PhasorMode=off  PhasorModeNumHarmonics=1  ConsistencySolver=NEWTON_XTOL_AFTER_FTOL  IndexReductionMethod=DerivativeReplacement  DoDC=off  ResidualTolerance=1e-09  ConsistencyTolSource=GLOBAL  ConsistencyAbsTol=0.001  ConsistencyRelTol=0.001  ConsistencyTolFactor=0.001  UseLocalSolver=off  LocalSolverChoice=NE_BACKWARD_EULER_ADVANCER  ResolveIndetEquations=on  FunctionEvalNumThread=1  LocalSolverSampleTime=0.01  DoFixedCost=off  MaxNonlinIter=3  MaxModeIter=2  ComputeImpulses=off  ImpulseIterations=2  LinearAlgebra=auto  LinearAlgebraNumThread=0  EquationFormulation=NE_TIME_EF  DelaysMemoryBudget=1024  AutomaticFiltering=on  FilteringTimeConstant=0.001  PartitionStorageMethod=AS_NEEDED  PartitionMemoryBudget=1024  PartitionMethod=ROBUST  MultibodyUseLocalSolver=off  MultibodyLocalSolverChoice=ODE1  MultibodyLocalSolverSampleTime=0.001
  Tires FL : sdl_lib/Tires & Vehicles/Tire (Magic Formula)  parameterization=sdl.enum.magic_tire_model.peak  F_z1=3000 N  F_x1=3500 N  kappa1=10  B_m=10  C_m=1.9  D_m=1  E_m=0.97  fz0=4000 N  p_Cx=1.685  p_Dx=[1.21, -.037]  p_Ex=[.344, .095, -.02, 0]  p_Kx=[21.51, -.163, .245]  p_Hx=[-.002, .002]  p_Vx=[0, 0]  rolling_radius_model=sdl.enum.RollingRadiusParameterization.Constant  r_e=tireRad m  r_0=0.3 m  breff=8.39  dreff=0.26  freff=0.074  q_re0=0.99  q_v1=0.008  longvl=17 m/s  cz=5e5 N/m  model_resistance=true  resistance_model=sdl.enum.rollingResistanceParameterization.constant  coeff=Veh.tirecR  p_tire=250e3 Pa  alpha=-0.003  beta=0.97  coeff_a=84e-4  coeff_b=6.2e-4 s/m  coeff_c=1.6e-4 s^2/m^2  p_tire0=240e3 Pa  fz0_resistance=4000 N  vH0=16 m/s  q_Sy=[.0082, 0, .0014, .001, 0, 0, 1.08, -.5]  v_thr=0.1 m/s  enable_scaling_coefficients=false  lfzO=1  lcx=1  lmux=1  lex=1  lkx=1  lhx=1  lvx=1  lmy=1  model_compliance=sdl.enum.compliance.off  stiffness=1e6 N/m  damping=1000 N*s/m  model_inertia=sdl.enum.model_inertia.on  inertia=tireInert kg*m^2  initial_velocity=0 rad/s  vxlow=1 m/s  v_tr_thr=0.1 m/s  kpumin=-1.5  kpumax=1.5
  Tires FR : sdl_lib/Tires & Vehicles/Tire (Magic Formula)  parameterization=sdl.enum.magic_tire_model.peak  F_z1=3000 N  F_x1=3500 N  kappa1=10  B_m=10  C_m=1.9  D_m=1  E_m=0.97  fz0=4000 N  p_Cx=1.685  p_Dx=[1.21, -.037]  p_Ex=[.344, .095, -.02, 0]  p_Kx=[21.51, -.163, .245]  p_Hx=[-.002, .002]  p_Vx=[0, 0]  rolling_radius_model=sdl.enum.RollingRadiusParameterization.Constant  r_e=tireRad m  r_0=0.3 m  breff=8.39  dreff=0.26  freff=0.074  q_re0=0.99  q_v1=0.008  longvl=17 m/s  cz=5e5 N/m  model_resistance=true  resistance_model=sdl.enum.rollingResistanceParameterization.constant  coeff=Veh.tirecR  p_tire=250e3 Pa  alpha=-0.003  beta=0.97  coeff_a=84e-4  coeff_b=6.2e-4 s/m  coeff_c=1.6e-4 s^2/m^2  p_tire0=240e3 Pa  fz0_resistance=4000 N  vH0=16 m/s  q_Sy=[.0082, 0, .0014, .001, 0, 0, 1.08, -.5]  v_thr=0.1 m/s  enable_scaling_coefficients=false  lfzO=1  lcx=1  lmux=1  lex=1  lkx=1  lhx=1  lvx=1  lmy=1  model_compliance=sdl.enum.compliance.off  stiffness=1e6 N/m  damping=1000 N*s/m  model_inertia=sdl.enum.model_inertia.on  inertia=tireInert kg*m^2  initial_velocity=0 rad/s  vxlow=1 m/s  v_tr_thr=0.1 m/s  kpumin=-1.5  kpumax=1.5
  Tires RL : sdl_lib/Tires & Vehicles/Tire (Magic Formula)  parameterization=sdl.enum.magic_tire_model.peak  F_z1=3000 N  F_x1=3500 N  kappa1=10  B_m=10  C_m=1.9  D_m=1  E_m=0.97  fz0=4000 N  p_Cx=1.685  p_Dx=[1.21, -.037]  p_Ex=[.344, .095, -.02, 0]  p_Kx=[21.51, -.163, .245]  p_Hx=[-.002, .002]  p_Vx=[0, 0]  rolling_radius_model=sdl.enum.RollingRadiusParameterization.Constant  r_e=tireRad m  r_0=0.3 m  breff=8.39  dreff=0.26  freff=0.074  q_re0=0.99  q_v1=0.008  longvl=17 m/s  cz=5e5 N/m  model_resistance=true  resistance_model=sdl.enum.rollingResistanceParameterization.constant  coeff=Veh.tirecR  p_tire=250e3 Pa  alpha=-0.003  beta=0.97  coeff_a=84e-4  coeff_b=6.2e-4 s/m  coeff_c=1.6e-4 s^2/m^2  p_tire0=240e3 Pa  fz0_resistance=4000 N  vH0=16 m/s  q_Sy=[.0082, 0, .0014, .001, 0, 0, 1.08, -.5]  v_thr=0.1 m/s  enable_scaling_coefficients=false  lfzO=1  lcx=1  lmux=1  lex=1  lkx=1  lhx=1  lvx=1  lmy=1  model_compliance=sdl.enum.compliance.off  stiffness=1e6 N/m  damping=1000 N*s/m  model_inertia=sdl.enum.model_inertia.on  inertia=tireInert kg*m^2  initial_velocity=0 rad/s  vxlow=1 m/s  v_tr_thr=0.1 m/s  kpumin=-1.5  kpumax=1.5
  Tires RR : sdl_lib/Tires & Vehicles/Tire (Magic Formula)  parameterization=sdl.enum.magic_tire_model.peak  F_z1=3000 N  F_x1=3500 N  kappa1=10  B_m=10  C_m=1.9  D_m=1  E_m=0.97  fz0=4000 N  p_Cx=1.685  p_Dx=[1.21, -.037]  p_Ex=[.344, .095, -.02, 0]  p_Kx=[21.51, -.163, .245]  p_Hx=[-.002, .002]  p_Vx=[0, 0]  rolling_radius_model=sdl.enum.RollingRadiusParameterization.Constant  r_e=tireRad m  r_0=0.3 m  breff=8.39  dreff=0.26  freff=0.074  q_re0=0.99  q_v1=0.008  longvl=17 m/s  cz=5e5 N/m  model_resistance=true  resistance_model=sdl.enum.rollingResistanceParameterization.constant  coeff=Veh.tirecR  p_tire=250e3 Pa  alpha=-0.003  beta=0.97  coeff_a=84e-4  coeff_b=6.2e-4 s/m  coeff_c=1.6e-4 s^2/m^2  p_tire0=240e3 Pa  fz0_resistance=4000 N  vH0=16 m/s  q_Sy=[.0082, 0, .0014, .001, 0, 0, 1.08, -.5]  v_thr=0.1 m/s  enable_scaling_coefficients=false  lfzO=1  lcx=1  lmux=1  lex=1  lkx=1  lhx=1  lvx=1  lmy=1  model_compliance=sdl.enum.compliance.off  stiffness=1e6 N/m  damping=1000 N*s/m  model_inertia=sdl.enum.model_inertia.on  inertia=tireInert kg*m^2  initial_velocity=0 rad/s  vxlow=1 m/s  v_tr_thr=0.1 m/s  kpumin=-1.5  kpumax=1.5
  Transfer Fcn : TransferFcn  Denominator=[0.01 1]
  Valve : autolibutils/Cont LPF  wc=125.66  AbsoluteTolerance=auto  aMode=6
  Vehicle : sdl_lib/Tires & Vehicles/Vehicle Body  mass=vehMass kg  n_w=Veh.numWheel  x_f=Veh.CGFA m  x_r=Veh.CGRA m  y_c=Veh.CGGround m  mass_var=simscape.enum.onoff.on  g=9.81 m/s^2  liftoff_warning=simscape.enum.onoff.on  area="Veh.AVeh    m^2"  Cd_var=false  Cd=Veh.cD  rho=1.18 kg/m^3  model_pitch=simscape.enum.onoff.off  inertia=4000 kg*m^2  suspension_model=sdl.enum.linearTLU.linear  k_f=1e4 N/m  b_f=1e4 N*s/m  k_r=1e4 N/m  b_r=1e4 N*s/m  k_f_TLU=[-2000, -1000, 0, 1000, 2000] N  x_f_TLU=[-.4, -.2, 0, .2, .4] m  b_f_TLU=[-200, -100, 0, 100, 200] N  v_f_TLU=[-4, -2, 0, 2, 4] m/s  k_r_TLU=[-2000, -1000, 0, 1000, 2000] N  x_r_TLU=[-.4, -.2, 0, .2, .4] m  b_r_TLU=[-200, -100, 0, 100, 200] N  v_r_TLU=[-4, -2, 0, 2, 4] m/s  interp_method=simscape.enum.interpolation.linear  extrap_method=simscape.enum.extrapolation.linear  model_hardstop=simscape.enum.onoff.off  upper_bound_f=.25 m  lower_bound_f=-.25 m  stop_k_f=1e6 N/m  stop_b_f=150 N*s/m  upper_bound_r=.25 m  lower_bound_r=-.25 m  stop_k_r=1e6 N/m  stop_b_r=150 N*s/m  initial_pitch=0 rad  initial_pitch_rate=0 rad/s  v_specify=on  v_priority=High  v=0 m/s  v_nominal_specify=off  v_nominal_value=1  v_nominal_unit=m/s
      settings: InternalSimscapePortConfiguration="{\"Bottom\":[{\"id\":\"NR\",\"label\":\"NR\",\"type\":\"output\"},{\"id\":\"NF\",\"label\":\"NF\",\"type\":\"output\"},{\"id\":\"beta\",\"label\":\"beta\",\"type\":\"input\"}],\"Left\":[{\"id\":\"H\",\"label\":\"H\",\"type\":\"foundation.mechanical.translational.translational\"}],\"Right\":[],\"Top\":[{\"id\":\"V\",\"label\":\"V\",\"type\":\"output\"},{\"id\":\"wind\",\"label\":\"W\",\"type\":\"input\"},{\"id\":\"cg_load\",\"label\":\"CG\",\"type\":\"input\"},{\"id\":\"mass_load\",\"label\":\"M\",\"type\":\"input\"}]}"
  Wind : fl_lib/Physical Signals/Sources/PS Constant  constant=0 m/s
  RA : PMIOPort  Side=Right
  tag scope: vehSpeed=global
  wires:
  Passenger mass/1(Out1) -> Simulink-PS Converter/1
  PS-Simulink Converter/1 -> Transfer Fcn/1  "VehSpd"
  Transfer Fcn/1 -> [vehSpeed]
  Dead Zone/1 -> Valve/1
  Valve/1 -> Product/2  "Flow"
  Product/1 -> Gain4/1
  Front Bias/1 -> Mux/2, Mux/1
  [cmd_brakes] -> Dead Zone/1
  Rear Bias/1 -> Mux/3, Mux/4
  Mux/1 -> Product/1
  Gain4/1 -> Selector3/1, Selector6/1, Selector1/1, Selector2/1
  Selector3/1 -> [cmd_brake_FR]
  Selector6/1 -> [cmd_brake_FL]
  [cmd_brake_FL] -> Simulink-PS Converter3/1
  [cmd_brake_FR] -> Simulink-PS Converter5/1
  Selector1/1 -> [cmd_brake_RR]
  [cmd_brake_RR] -> Simulink-PS Converter4/1
  Selector2/1 -> [cmd_brake_RL]
  [cmd_brake_RL] -> Simulink-PS Converter2/1
  connections:
  Disc Brake - Front L/LConn2 -- Tires FL/LConn2
  Tires FR/LConn2 -- Disc Brake - Front R/LConn2
  Tires FR/RConn2 -- Solver Configuration/RConn1 -- Tires RL/RConn2 -- Tires FL/RConn2 -- Tires RR/RConn2 -- PWRS6/RConn1
  Vehicle/RConn2 -- Tires FL/LConn1 -- Tires FR/LConn1
  PWRS6/LConn1 -- Vehicle/LConn1
  Simulink-PS Converter/RConn1 -- Vehicle/LConn5
  Wind/RConn1 -- Vehicle/LConn3
  Road Incline/RConn1 -- Vehicle/RConn3
  Vehicle/RConn1 -- Tires RL/LConn1 -- Tires RR/LConn1
  PS-Simulink Converter/LConn1 -- Vehicle/LConn2
  Disc Brake - Rear L/LConn2 -- Differential/RConn1 -- Tires RL/LConn2
  Disc Brake - Rear R/LConn1 -- Simulink-PS Converter4/RConn1
  Disc Brake - Front L/LConn1 -- Simulink-PS Converter3/RConn1
  Simulink-PS Converter5/RConn1 -- Disc Brake - Front R/LConn1
  Differential/LConn1 -- RA/RConn1
  Disc Brake - Rear R/LConn2 -- Tires RR/LConn2 -- Differential/RConn2
  Simulink-PS Converter2/RConn1 -- Disc Brake - Rear L/LConn1

== system BEV_Thermal_Management/EV1 ==
  Evaporator Expansion Valve : SimscapeFluids_lib/Two-Phase Fluid/Valves & Orifices/Flow Control Valves/Thermostatic Expansion Valve (2P)  valve_parameterization=fluids.two_phase_fluid.valves_orifices.flow_control_valves.enum.ThermostaticExpansionValveParameterization.Nominal  capacity_spec=fluids.two_phase_fluid.valves_orifices.flow_control_valves.enum.ThermostaticExpansionValveCapacitySpec.HeatTransfer  Q_nominal=2000 W  Q_max=4000 W  mdot_nominal=0.005 kg/s  mdot_max=0.008 kg/s  pressure_spec=fluids.two_phase_fluid.valves_orifices.flow_control_valves.enum.ThermostaticExpansionValvePressureSpec.SaturationTemperature  p_cond_nominal=1.5 MPa  p_evap_nominal=0.5 MPa  T_cond_nominal=40 degC  T_evap_nominal=1 degC  delta_T_sub=5 deltaK  delta_T_nominal=10 deltaK  delta_T_static=5 deltaK  mop=fluids.two_phase_fluid.valves_orifices.flow_control_valves.enum.ThermostaticExpansionValveMOP.Off  p_mop=0.5 MPa  T_mop=288.15 K  T_evap_out_TLU1=0 : 10 : 40 degC  p_bulb_TLU1=0.3 : 0.1 : 0.7 MPa  lift_TLU2=0 : 0.15 : 0.6 mm  p_evap_TLU2=0.3 : -0.05 : 0.1 MPa  lift_TLU3=0 : 0.15 : 0.6 mm  mdot_TLU3=0 : 0.015 : 0.06 kg/s  p_cond_ref=2 MPa  p_evap_ref=0.2 MPa  T_evap_out_ref=0 degC  delta_T_sub_ref=5 deltaK  pressure_equalization=fluids.two_phase_fluid.valves_orifices.flow_control_valves.enum.ThermostaticExpansionValveEqualization.External  bulb_dynamics=simscape.enum.onoff.off  tau_bulb=20 s  leakage_fraction=1e-6  smoothing_factor=0.01  B_lam=0.999  tau_x=0.1 s  area=pi * refrigerant_pipe_D^2 / 4 m^2
      settings: InternalSimscapePortConfiguration="{\"Bottom\":[],\"Left\":[{\"id\":\"A\",\"label\":\"A\",\"type\":\"foundation.two_phase_fluid.two_phase_fluid\"}],\"Right\":[{\"id\":\"B\",\"label\":\"B\",\"type\":\"foundation.two_phase_fluid.two_phase_fluid\"}],\"Top\":[{\"id\":\"S\",\"label\":\"S\",\"type\":\"foundation.two_phase_fluid.two_phase_fluid\"},{\"id\":\"E\",\"label\":\"E\",\"type\":\"foundation.two_phase_fluid.two_phase_fluid\"}]}"
  Simscape Bus : SimscapeBus  HierarchyStrings=bulb;outlet
  B : PMIOPort  Side=Left
  A : PMIOPort  Port=2  Side=Right
  connections:
  Evaporator Expansion Valve/LConn1 -- A/RConn1
  Evaporator Expansion Valve/LConn2 -- Simscape Bus/LConn1 -- Evaporator Expansion Valve/LConn3
  Evaporator Expansion Valve/RConn1 -- Simscape Bus/LConn2
  B/RConn1 -- Simscape Bus/RConn1
